simulink model "PID_correection_ideal_parametertest"  (R2025a)
settings: Solver=ode4  StartTime=0.0  StopTime=inf  FixedStep=0.0001  RelTol=1e-3  EnableMultiTasking=on
InitFcn:
  | addpath('functions');
model workspace (MATLAB code in the model file):
  | arm_torque = 0;
  | L_arm = 0.115;
  | I_arm = 6.5e-4;
  | lcom_1 = 0.058;
  | I_1 = 3.7e-5;
  | m_1 = 0.023;
  | L_1 = 0.13;
  | 
  | init_cond = [pi/2; 0; 0.26; 0];
undefined symbols (not defined in the file or in its folder): DiscIntNeverNeededParam, Ts
libraries: slpidlib x2
settings Model: PacingRate=0.400000  Creator=Esther  LastModifiedBy=marcus
settings SolverCC: AutoInsertRateTranBlk=on
settings OptimizationCC: DefaultParameterBehavior=Inlined  EnhancedBackFolding=on  PassReuseOutputArgsAs=Individual arguments  ZeroExternalMemoryAtStartup=off  ZeroInternalMemoryAtStartup=off  MaxStackSize=64  OptimizeBlockOrder=speed  DifferentSizesBufferReuse=on  OptimizationCustomize=off  EfficientTunableParamExpr=on
settings DebuggingCC: ParameterTunabilityLossMsg=error
settings HardwareCC: ProdBitPerPointer=32.0  ProdBitPerSizeT=32.0  ProdBitPerPtrDiffT=32.0  ProdLargestAtomicInteger=Long  ProdLargestAtomicFloat=Double  ProdWordSize=32.0  ProdLongLongMode=on  ProdHWDeviceType=ARM Compatible->ARM Cortex-M
settings RTWCC: SystemTargetFile=ert.tlc  TemplateMakefile=ert_default_tmf  Toolchain=Armclang Compiler  Description=Embedded Coder
settings CodeAppCC: ForceParamTrailComments=on  IgnoreCustomStorageClasses=off  OperatorAnnotations=on  SimulinkDataObjDesc=on  SFDataObjDesc=on  InsertBlockDesc=on
settings ERTTargetCC: ExtModeTransport=3.0  ExtModeStaticAllocSize=2048.0  ERTCustomFileTemplate=example_file_process.tlc  TargetLangStandard=C99 (ISO)  CodeReplacementLibrary=ARM Cortex-M

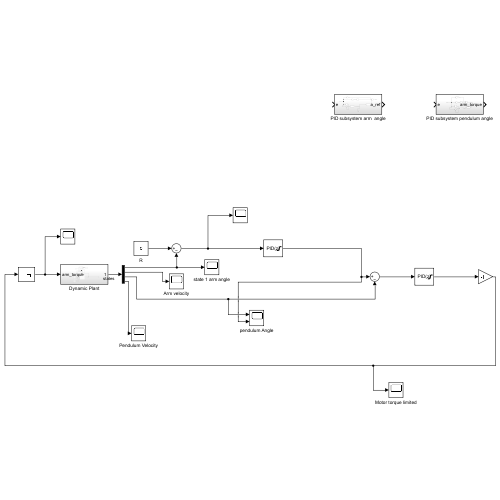
[thumbnail: Simulink's stored preview of the top-level diagram]
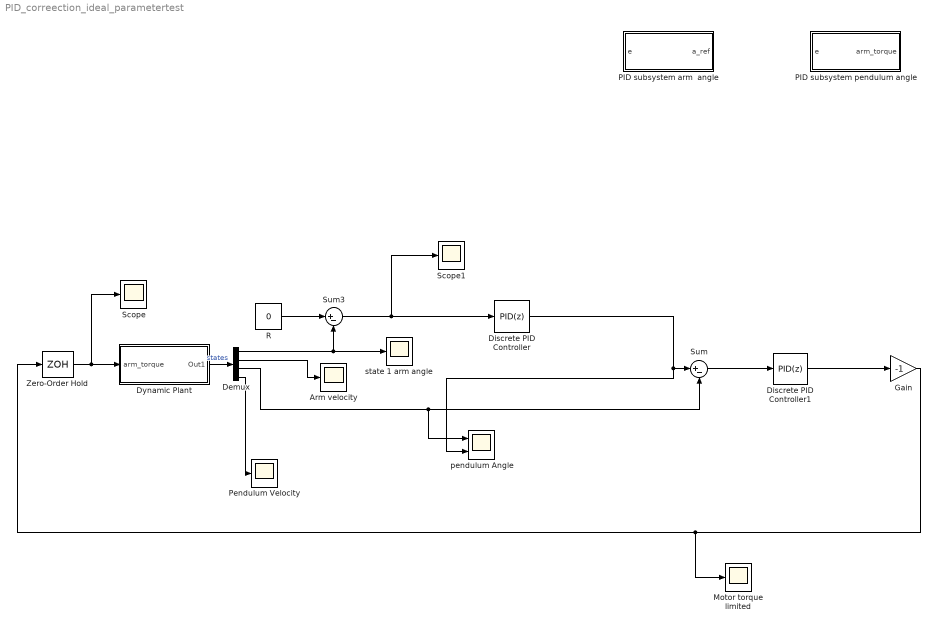
== system PID_correection_ideal_parametertest ==
  Arm velocity : Scope
      settings: ActiveDisplayYMinimum=-2.9332109336231191  ActiveDisplayYMaximum=4.428663277226133  DataLoggingVariableName=ScopeData4
  Demux : Demux
  Discrete PID Controller : slpidlib/PID Controller  Controller=PID  Form=Parallel  TimeDomain=Discrete-time  UseExternalTs=off  SampleTime=Ts  IntegratorMethod=Forward Euler  FilterMethod=Forward Euler  ControllerParametersSource=internal  P=0.05  I=0  UseKiTs=on  D=0.08  UseExternalDerivativeSource=off  N=8  UseFilter=on  TunerSelectOption=Transfer Function Based (PID Tuner App)  InitialConditionSource=internal  InitialConditionForIntegrator=0  InitialConditionForFilter=0  DifferentiatorICPrevScaledInput=0  ExternalReset=none  TrackingMode=off  Kt=1  LimitOutput=on  SatLimitsSource=internal  UpperSaturationLimit=0.1  LowerSaturationLimit=-0.1  LinearizeAsGain=off  AntiWindupMode=none  Kb=1  LimitIntegrator=off  UpperIntegratorSaturationLimit=inf  LowerIntegratorSaturationLimit=-inf  POutMin=[]  POutMax=[]  IOutMin=[]  IOutMax=[]  DOutMin=[]  DOutMax=[]  NOutMin=[]  NOutMax=[]  SumOutMin=[]  SumOutMax=[]  SaturationOutMin=[]  SaturationOutMax=[]  PParamMin=[]  PParamMax=[]  IParamMin=[]  IParamMax=[]  DParamMin=[]  DParamMax=[]  NParamMin=[]  NParamMax=[]  KbParamMin=[]  KbParamMax=[]  KtParamMin=[]  KtParamMax=[]  KbOutMin=[]  KbOutMax=[]  KtOutMin=[]  KtOutMax=[]  IntegratorOutMin=[]  IntegratorOutMax=[]  FilterOutMin=[]  FilterOutMax=[]  SumI1OutMin=[]  SumI1OutMax=[]  SumI2OutMin=[]  SumI2OutMax=[]  SumI3OutMin=[]  SumI3OutMax=[]  SumI4OutMin=[]  SumI4OutMax=[]  SumDOutMin=[]  SumDOutMax=[]  DifferentiatorOutMin=[]  DifferentiatorOutMax=[]  FilterDiffOutCoefMin=[]  FilterDiffOutCoefMax=[]  ReciprocalOutMin=[]  ReciprocalOutMax=[]  SumDenOutMin=[]  SumDenOutMax=[]  SumNumOutMin=[]  SumNumOutMax=[]  DivideOutMin=[]  DivideOutMax=[]  UdiffTsProdOutMin=[]  UdiffTsProdOutMax=[]  NTsProdOutMin=[]  NTsProdOutMax=[]  UintegralTsProdOutMin=[]  UintegralTsProdOutMax=[]  UngainTsProdOutMin=[]  UngainTsProdOutMax=[]  ClampingZeroOutDataTypeStr=Inherit: Inherit via back propagation  ClampingZeroOutMin=[]  ClampingZeroOutMax=[]  FilterDenConstantOutDataTypeStr=Inherit: Inherit via back propagation  FilterDenConstantOutMin=[]  FilterDenConstantOutMax=[]  PCopyOutDataTypeStr=Inherit: Inherit via back propagation  PCopyOutMin=[]  PCopyOutMax=[]  NCopyOutDataTypeStr=Inherit: Inherit via back propagation  NCopyOutMin=[]  NCopyOutMax=[]  IntegratorContinuousStateAttributes=''  IntegratorStateMustResolveToSignalObject=off  IntegratorRTWStateStorageClass=Auto  FilterContinuousStateAttributes=''  FilterStateMustResolveToSignalObject=off  FilterRTWStateStorageClass=Auto  ParallelPVariant=InternalParameters  IdealPVariant=Disabled  IVariant=InternalParameters  DVariant=InternalParameters  IntegratorVariant=Discrete  SatVariant=Enabled  AWVariant=Passthrough  PCopyVariant=Disabled  TRVariant=Disabled  FdbkBlocksVariant=Forward  IdealPFdbkVariant=Disabled  SatFdbkVariant=Disabled  DerivativeFilterVariant=ForwardEulerFilter  NVariant=InternalParameters  NCopyVariant=Disabled  FilterICVariant=InternalICsFilter  IntegratorICVariant=InternalICs  ExternalResetVariant=Disabled  TRSumVariant=Passthrough  SumFdbkVariant=Disabled  SumVariant=Sum_PID  TsampFilterVariant=InternalTs  TsampNgainVariant=Passthrough  TsampIntegralVariant=Disabled_SignalSpec  ExternalSaturationOutDataTypeStr=Inherit: Same as second input  DerivativeSourceVariant=ErrorSignal  PreIntVariant=InternalPreInt
      settings: LibrarySourceBlock=simulink/Discrete/Discrete PID Controller
  Discrete PID Controller1 : slpidlib/PID Controller  Controller=PID  Form=Parallel  TimeDomain=Discrete-time  UseExternalTs=off  SampleTime=Ts  IntegratorMethod=Forward Euler  FilterMethod=Forward Euler  ControllerParametersSource=internal  P=60  I=0  UseKiTs=on  D=2  UseExternalDerivativeSource=off  N=50  UseFilter=on  TunerSelectOption=Transfer Function Based (PID Tuner App)  InitialConditionSource=internal  InitialConditionForIntegrator=0  InitialConditionForFilter=0  DifferentiatorICPrevScaledInput=0  ExternalReset=none  TrackingMode=off  Kt=1  LimitOutput=on  SatLimitsSource=internal  UpperSaturationLimit=0.088  LowerSaturationLimit=-0.088  LinearizeAsGain=off  AntiWindupMode=clamping  Kb=1  LimitIntegrator=off  UpperIntegratorSaturationLimit=inf  LowerIntegratorSaturationLimit=-inf  POutMin=[]  POutMax=[]  IOutMin=[]  IOutMax=[]  DOutMin=[]  DOutMax=[]  NOutMin=[]  NOutMax=[]  SumOutMin=[]  SumOutMax=[]  SaturationOutMin=[]  SaturationOutMax=[]  PParamMin=[]  PParamMax=[]  IParamMin=[]  IParamMax=[]  DParamMin=[]  DParamMax=[]  NParamMin=[]  NParamMax=[]  KbParamMin=[]  KbParamMax=[]  KtParamMin=[]  KtParamMax=[]  KbOutMin=[]  KbOutMax=[]  KtOutMin=[]  KtOutMax=[]  IntegratorOutMin=[]  IntegratorOutMax=[]  FilterOutMin=[]  FilterOutMax=[]  SumI1OutMin=[]  SumI1OutMax=[]  SumI2OutMin=[]  SumI2OutMax=[]  SumI3OutMin=[]  SumI3OutMax=[]  SumI4OutMin=[]  SumI4OutMax=[]  SumDOutMin=[]  SumDOutMax=[]  DifferentiatorOutMin=[]  DifferentiatorOutMax=[]  FilterDiffOutCoefMin=[]  FilterDiffOutCoefMax=[]  ReciprocalOutMin=[]  ReciprocalOutMax=[]  SumDenOutMin=[]  SumDenOutMax=[]  SumNumOutMin=[]  SumNumOutMax=[]  DivideOutMin=[]  DivideOutMax=[]  UdiffTsProdOutMin=[]  UdiffTsProdOutMax=[]  NTsProdOutMin=[]  NTsProdOutMax=[]  UintegralTsProdOutMin=[]  UintegralTsProdOutMax=[]  UngainTsProdOutMin=[]  UngainTsProdOutMax=[]  ClampingZeroOutDataTypeStr=Inherit: Inherit via back propagation  ClampingZeroOutMin=[]  ClampingZeroOutMax=[]  FilterDenConstantOutDataTypeStr=Inherit: Inherit via back propagation  FilterDenConstantOutMin=[]  FilterDenConstantOutMax=[]  PCopyOutDataTypeStr=Inherit: Inherit via back propagation  PCopyOutMin=[]  PCopyOutMax=[]  NCopyOutDataTypeStr=Inherit: Inherit via back propagation  NCopyOutMin=[]  NCopyOutMax=[]  IntegratorContinuousStateAttributes=''  IntegratorStateMustResolveToSignalObject=off  IntegratorRTWStateStorageClass=Auto  FilterContinuousStateAttributes=''  FilterStateMustResolveToSignalObject=off  FilterRTWStateStorageClass=Auto  ParallelPVariant=InternalParameters  IdealPVariant=Disabled  IVariant=InternalParameters  DVariant=InternalParameters  IntegratorVariant=Discrete  SatVariant=Enabled  AWVariant=DiscClampingParallel  PCopyVariant=Disabled  TRVariant=Disabled  FdbkBlocksVariant=Forward  IdealPFdbkVariant=Disabled  SatFdbkVariant=Disabled  DerivativeFilterVariant=ForwardEulerFilter  NVariant=InternalParameters  NCopyVariant=Disabled  FilterICVariant=InternalICsFilter  IntegratorICVariant=InternalICs  ExternalResetVariant=Disabled  TRSumVariant=Passthrough  SumFdbkVariant=Disabled  SumVariant=Sum_PID  TsampFilterVariant=InternalTs  TsampNgainVariant=Passthrough  TsampIntegralVariant=Disabled_SignalSpec  ExternalSaturationOutDataTypeStr=Inherit: Same as second input  DerivativeSourceVariant=ErrorSignal  PreIntVariant=InternalPreInt
      settings: LibrarySourceBlock=simulink/Discrete/Discrete PID Controller
  Dynamic Plant : Subsystem
  Gain : Gain  Gain=-1
  Motor torque limited : Scope
      settings: ActiveDisplayYMinimum=-0.10999999999999999  ActiveDisplayYMaximum=0.10999999999999999  DataLoggingVariableName=ScopeData5
  PID subsystem arm  angle : Subsystem
  PID subsystem pendulum angle : Subsystem
  Pendulum Velocity : Scope
      settings: ActiveDisplayYMinimum=-2.023298125624855  ActiveDisplayYMaximum=2.0235795712360787  DataLoggingVariableName=ScopeData2
  R : Constant  Value=0
  Scope : Scope
      settings: DataLoggingVariableName=ScopeData7
  Scope1 : Scope
      settings: ActiveDisplayYMinimum=-1  ActiveDisplayYMaximum=1  DataLoggingVariableName=ScopeData3
  Sum : Sum  Inputs=|+-
  Sum3 : Sum  Inputs=|+-
  Zero-Order Hold : ZeroOrderHold  SampleTime=-1
  pendulum Angle : Scope  NumInputPorts=2
      settings: ActiveDisplayYMinimum=-0.14582152994796849  ActiveDisplayYMaximum=0.30509128110532979  DataLoggingVariableName=ScopeData6
  state 1 arm angle : Scope
      settings: ActiveDisplayYMinimum=-0.33874782734308273  ActiveDisplayYMaximum=2.8578499042965384
  wires:
  Dynamic Plant/1(Out1) -> Demux/1  "states"
  R/1 -> Sum3/1
  Demux/4 -> Pendulum Velocity/1
  Demux/2 -> Arm velocity/1
  Zero-Order Hold/1 -> Scope/1, Dynamic Plant/1(arm_torque)
  Sum3/1 -> Scope1/1, Discrete PID Controller/1
  Gain/1 -> Zero-Order Hold/1, Motor torque limited/1
  Demux/1 -> Sum3/2, state 1 arm angle/1
  Demux/3 -> pendulum Angle/1, Sum/2
  Discrete PID Controller/1 -> pendulum Angle/2, Sum/1
  Sum/1 -> Discrete PID Controller1/1
  Discrete PID Controller1/1 -> Gain/1

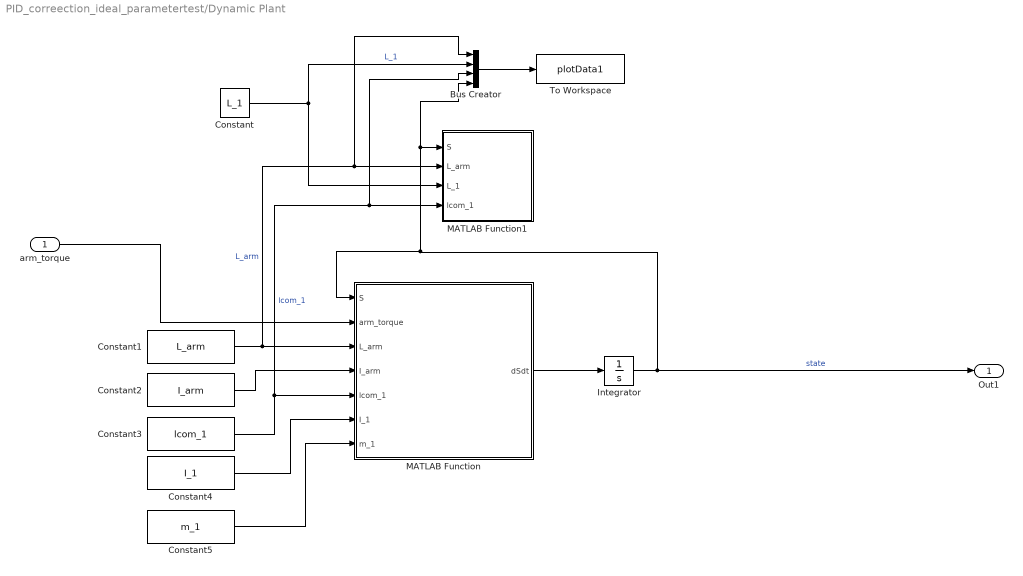
== system PID_correection_ideal_parametertest/Dynamic Plant ==
  arm_torque : Inport
  Bus Creator : BusCreator  Inputs=4
  Constant : Constant  Value=L_1
  Constant1 : Constant  Value=L_arm
  Constant2 : Constant  Value=I_arm
  Constant3 : Constant  Value=lcom_1
  Constant4 : Constant  Value=I_1
  Constant5 : Constant  Value=m_1
  Integrator : Integrator  InitialCondition=init_cond
  MATLAB Function : MATLAB Function  TreatAsAtomicUnit=on
  MATLAB Function1 : MATLAB Function  TreatAsAtomicUnit=on
  To Workspace : ToWorkspace  VariableName=plotData1  SaveFormat=Timeseries  SampleTime=-1
  Out1 : Outport
  wires:
  Bus Creator/1 -> To Workspace/1
  Constant/1 -> Bus Creator/2, MATLAB Function1/3(L_1)  "L_1"
  Constant2/1 -> MATLAB Function/4(I_arm)
  Constant4/1 -> MATLAB Function/6(I_1)
  Constant1/1 -> MATLAB Function/3(L_arm), Bus Creator/1, MATLAB Function1/2(L_arm)  "L_arm"
  Integrator/1 -> Out1/1, MATLAB Function/1(S), MATLAB Function1/1(S), Bus Creator/4  "state"
  Constant3/1 -> Bus Creator/3, MATLAB Function1/4(lcom_1), MATLAB Function/5(lcom_1)  "lcom_1"
  Constant5/1 -> MATLAB Function/7(m_1)
  arm_torque/1 -> MATLAB Function/2(arm_torque)
  MATLAB Function/1(dSdt) -> Integrator/1

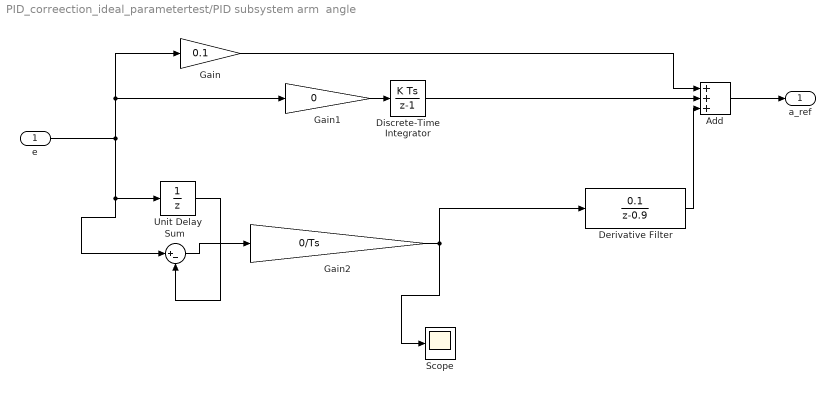
== system PID_correection_ideal_parametertest/PID subsystem arm  angle ==
  e : Inport
  Add : Sum  Inputs=+++
  Derivative Filter : DiscreteTransferFcn  Numerator=[0.1]  Denominator=[1 -0.9]
  Discrete-Time Integrator : DiscreteIntegrator  gainval=1  SampleTime=Ts  ICPrevOutput=DiscIntNeverNeededParam  ICPrevScaledInput=DiscIntNeverNeededParam
  Gain : Gain  Gain=0.1
  Gain1 : Gain  Gain=0
  Gain2 : Gain  Gain=0/Ts
  Scope : Scope
      settings: ActiveDisplayYMinimum=-1  ActiveDisplayYMaximum=1
  Sum : Sum  Inputs=|+-
  Unit Delay : UnitDelay  SampleTime=Ts  HasFrameUpgradeWarning=on
  a_ref : Outport
  wires:
  e/1 -> Gain/1, Gain1/1, Sum/1, Unit Delay/1
  Unit Delay/1 -> Sum/2
  Discrete-Time Integrator/1 -> Add/2
  Gain/1 -> Add/1
  Add/1 -> a_ref/1
  Gain1/1 -> Discrete-Time Integrator/1
  Sum/1 -> Gain2/1
  Gain2/1 -> Derivative Filter/1, Scope/1
  Derivative Filter/1 -> Add/3

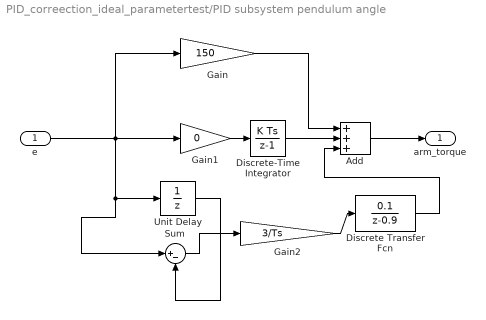
== system PID_correection_ideal_parametertest/PID subsystem pendulum angle ==
  e : Inport
  Add : Sum  Inputs=+++
  Discrete Transfer Fcn : DiscreteTransferFcn  Numerator=[0.1]  Denominator=[1 -0.9]
  Discrete-Time Integrator : DiscreteIntegrator  gainval=1  SampleTime=Ts  ICPrevOutput=DiscIntNeverNeededParam  ICPrevScaledInput=DiscIntNeverNeededParam
  Gain : Gain  Gain=150
  Gain1 : Gain  Gain=0
  Gain2 : Gain  Gain=3/Ts
  Sum : Sum  Inputs=|+-
  Unit Delay : UnitDelay  SampleTime=Ts  HasFrameUpgradeWarning=on
  arm_torque : Outport
  wires:
  e/1 -> Sum/1, Unit Delay/1, Gain/1, Gain1/1
  Unit Delay/1 -> Sum/2
  Discrete-Time Integrator/1 -> Add/2
  Gain/1 -> Add/1
  Add/1 -> arm_torque/1
  Gain1/1 -> Discrete-Time Integrator/1
  Sum/1 -> Gain2/1
  Gain2/1 -> Discrete Transfer Fcn/1
  Discrete Transfer Fcn/1 -> Add/3

== matlab function PID_correection_ideal_parametertest/Dynamic Plant/MATLAB Function ==
  data: S input size=4; dSdt output size=4; arm_torque input size=1; L_arm input size=1; I_arm input size=1; lcom_1 input size=1; I_1 input size=1; m_1 input size=1
function dSdt = get_dSdt(S, arm_torque, L_arm, I_arm, lcom_1, I_1, m_1)
    t = 0;
    g = 9.81;
    phys_param = [L_arm, I_arm, lcom_1, I_1, m_1, g];
    fric_arm = [0.018, 0.018, 100];
    fric_1 = [0.0001, 0.0001, 100];
    dSdt = furuta_single_state_derivative(t, S, arm_torque, phys_param, fric_arm, fric_1);
end

== matlab function PID_correection_ideal_parametertest/Dynamic Plant/MATLAB Function1 ==
  settings: updateMethod=DISCRETE
  data: S input; L_arm input; L_1 input; lcom_1 input
function animation(S, L_arm, L_1, lcom_1)
    update_ratio = 100;
    realtime_animation_single(S, L_arm, L_1, lcom_1, update_ratio);
end
